simulink model "trt_model"  (R2025a)
settings: Solver=ode4  StartTime=0.0  StopTime=100  FixedStep=P.dt_sim  RelTol=1e-3
values from neighbouring files (symbols this model uses):
  C = aggressive_bypass_tuning(P, C, 0.3); end    [make_scenario.m]
  P = params()    [run_scenarios.m]
undefined symbols (not defined in the file or in its folder): X0
settings Model: Creator=andreazanelli  LastModifiedBy=andreazanelli
settings DataIOCC: SaveOutput=off  SignalLogging=off  SaveTime=off
settings DebuggingCC: AlgebraicLoopMsg=error

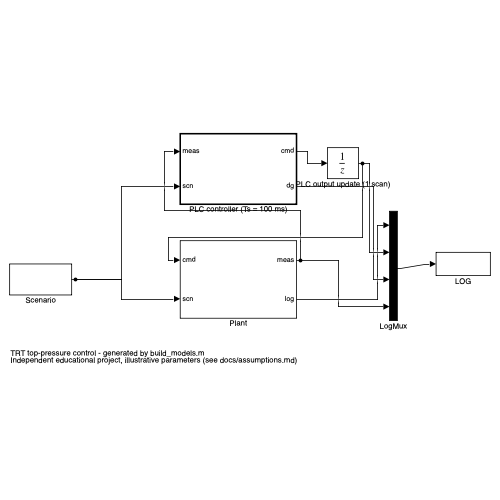
[thumbnail: Simulink's stored preview of the top-level diagram]
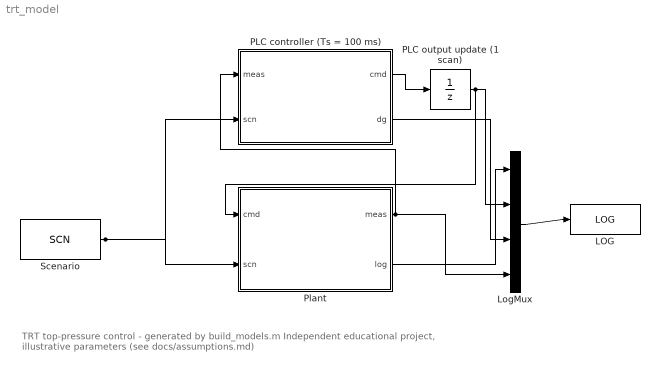
== system trt_model ==
  note: TRT top-pressure control - generated by build_models.m
      | Independent educational project, illustrative parameters (see docs/assumptions.md)
  LOG : ToWorkspace  VariableName=LOG  SaveFormat=Structure With Time  SampleTime=0.05
  LogMux : Mux
  PLC controller (Ts = 100 ms) : Subsystem  TreatAsAtomicUnit=on  SystemSampleTime=C.Ts
  PLC output update (1 scan) : UnitDelay  InitialCondition=C.init.cmd  SampleTime=C.Ts  HasFrameUpgradeWarning=on
  Plant : Subsystem
  Scenario : FromWorkspace  VariableName=SCN  SampleTime=C.Ts  Interpolate=off  OutputAfterFinalValue=Holding final value
  wires:
  Scenario/1 -> Plant/2(scn), PLC controller (Ts = 100 ms)/2(scn)
  PLC controller (Ts = 100 ms)/1(cmd) -> PLC output update (1 scan)/1
  PLC output update (1 scan)/1 -> Plant/1(cmd), LogMux/2
  Plant/1(meas) -> PLC controller (Ts = 100 ms)/1(meas), LogMux/4
  Plant/2(log) -> LogMux/1
  PLC controller (Ts = 100 ms)/2(dg) -> LogMux/3
  LogMux/1 -> LOG/1

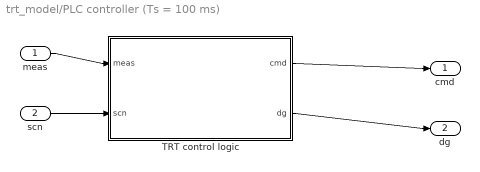
== system trt_model/PLC controller (Ts = 100 ms) ==
  meas : Inport
  scn : Inport  Port=2
  TRT control logic : MATLAB Function  TreatAsAtomicUnit=on
  cmd : Outport
  dg : Outport  Port=2
  wires:
  meas/1 -> TRT control logic/1(meas)
  scn/1 -> TRT control logic/2(scn)
  TRT control logic/1(cmd) -> cmd/1
  TRT control logic/2(dg) -> dg/1

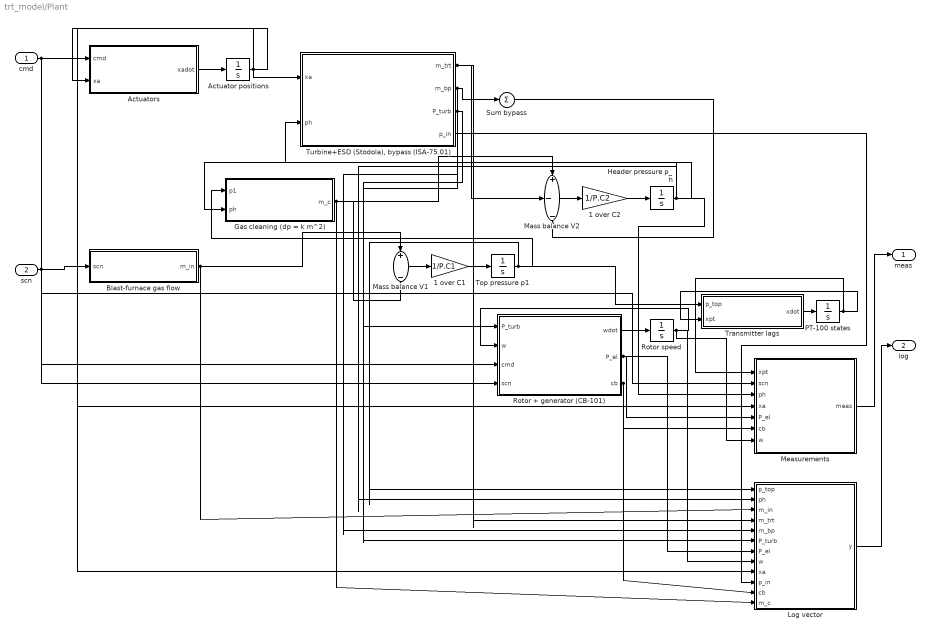
== system trt_model/Plant ==
  cmd : Inport
  scn : Inport  Port=2
  1 over C1 : Gain  Gain=1/P.C1
  1 over C2 : Gain  Gain=1/P.C2
  Actuator positions : Integrator  InitialCondition=X0.xa  LimitOutput=on  UpperSaturationLimit=1  LowerSaturationLimit=0
  Actuators : MATLAB Function  TreatAsAtomicUnit=on
  Blast-furnace gas flow : MATLAB Function  TreatAsAtomicUnit=on
  Gas cleaning (dp = k m^2) : MATLAB Function  TreatAsAtomicUnit=on
  Header pressure p_h : Integrator  InitialCondition=X0.ph
  Log vector : MATLAB Function  TreatAsAtomicUnit=on
  Mass balance V1 : Sum  Inputs=+-
  Mass balance V2 : Sum  Inputs=+--
  Measurements : MATLAB Function  TreatAsAtomicUnit=on
  PT-100 states : Integrator  InitialCondition=X0.xpt
  Rotor + generator (CB-101) : MATLAB Function  TreatAsAtomicUnit=on
  Rotor speed : Integrator  InitialCondition=X0.w
  Sum bypass : Sum  Inputs=+
  Top pressure p1 : Integrator  InitialCondition=X0.p1
  Transmitter lags : MATLAB Function  TreatAsAtomicUnit=on
  "Turbine+ESD (Stodola), bypass (ISA-75.01)" : MATLAB Function  TreatAsAtomicUnit=on
  meas : Outport
  log : Outport  Port=2
  wires:
  cmd/1 -> Actuators/1(cmd), Rotor + generator (CB-101)/3(cmd)
  Actuator positions/1 -> Actuators/2(xa), "Turbine+ESD (Stodola), bypass (ISA-75.01)"/1(xa), Measurements/4(xa), Log vector/9(xa)
  Actuators/1(xadot) -> Actuator positions/1
  Header pressure p_h/1 -> "Turbine+ESD (Stodola), bypass (ISA-75.01)"/2(ph), Gas cleaning (dp = k m^2)/2(ph), Measurements/3(ph), Log vector/2(ph)
  scn/1 -> Blast-furnace gas flow/1(scn), Rotor + generator (CB-101)/4(scn), Measurements/2(scn)
  Top pressure p1/1 -> Gas cleaning (dp = k m^2)/1(p1), Transmitter lags/1(p_top), Log vector/1(p_top)
  Blast-furnace gas flow/1(m_in) -> Mass balance V1/1, Log vector/3(m_in)
  Gas cleaning (dp = k m^2)/1(m_c) -> Mass balance V1/2, Mass balance V2/1, Log vector/12(m_c)
  Mass balance V1/1 -> 1 over C1/1
  1 over C1/1 -> Top pressure p1/1
  "Turbine+ESD (Stodola), bypass (ISA-75.01)"/1(m_trt) -> Mass balance V2/2, Log vector/4(m_trt)
  "Turbine+ESD (Stodola), bypass (ISA-75.01)"/2(m_bp) -> Sum bypass/1, Log vector/5(m_bp)
  Sum bypass/1 -> Mass balance V2/3
  Mass balance V2/1 -> 1 over C2/1
  1 over C2/1 -> Header pressure p_h/1
  "Turbine+ESD (Stodola), bypass (ISA-75.01)"/3(P_turb) -> Rotor + generator (CB-101)/1(P_turb), Log vector/6(P_turb)
  Rotor speed/1 -> Rotor + generator (CB-101)/2(w), Measurements/7(w), Log vector/8(w)
  Rotor + generator (CB-101)/1(wdot) -> Rotor speed/1
  PT-100 states/1 -> Transmitter lags/2(xpt), Measurements/1(xpt)
  Transmitter lags/1(xdot) -> PT-100 states/1
  Rotor + generator (CB-101)/2(P_el) -> Measurements/5(P_el), Log vector/7(P_el)
  Rotor + generator (CB-101)/3(cb) -> Measurements/6(cb), Log vector/11(cb)
  Measurements/1(meas) -> meas/1
  "Turbine+ESD (Stodola), bypass (ISA-75.01)"/4(p_in) -> Log vector/10(p_in)
  Log vector/1(y) -> log/1

== matlab function trt_model/PLC controller (Ts = 100 ms)/TRT control logic ==
  data: meas input; cmd output; scn input; dg output; C parameter
function [cmd, dg] = f(meas, scn, C)
[cmd, dg] = trt_controller_step(meas, scn, C);

== matlab function trt_model/Plant/Turbine+ESD (Stodola), bypass (ISA-75.01) ==
  data: xa input; m_trt output; ph input; m_bp output; P_turb output; p_in output; P parameter
function [m_trt, m_bp, P_turb, p_in] = f(xa, ph, P)
[m_trt, m_bp, P_turb, p_in] = plant_flows(xa, ph, P);

== matlab function trt_model/Plant/Actuators ==
  data: cmd input; xadot output; xa input; P parameter
function xadot = f(cmd, xa, P)
xadot = plant_actuators(cmd, xa, P);

== matlab function trt_model/Plant/Blast-furnace gas flow ==
  data: scn input; m_in output
function m_in = f(scn)
m_in = scn(1);

== matlab function trt_model/Plant/Gas cleaning (dp = k m^2) ==
  data: p1 input; m_c output; ph input; P parameter
function m_c = f(p1, ph, P)
m_c = plant_cleaning(p1, ph, P);

== matlab function trt_model/Plant/Rotor + generator (CB-101) ==
  data: P_turb input; wdot output; w input; cmd input; scn input; P_el output; cb output; P parameter
function [wdot, P_el, cb] = f(P_turb, w, cmd, scn, P)
[wdot, P_el, cb] = plant_rotor(P_turb, w, cmd, scn, P);

== matlab function trt_model/Plant/Transmitter lags ==
  data: p_top input; xdot output; xpt input; P parameter
function xdot = f(p_top, xpt, P)
xdot = (p_top - xpt) / P.pt.tau;

== matlab function trt_model/Plant/Measurements ==
  data: xpt input; meas output; scn input; ph input; xa input; P_el input; cb input; w input; P parameter
function meas = f(xpt, scn, ph, xa, P_el, cb, w, P)
meas = plant_meas(xpt, scn, ph, xa, P_el, cb, w, P);

== matlab function trt_model/Plant/Log vector ==
  data: p_top input; y output; ph input; m_in input; m_trt input; m_bp input; P_turb input; P_el input; w input; xa input; p_in input; cb input; m_c input
function y = f(p_top, ph, m_in, m_trt, m_bp, P_turb, P_el, w, xa, p_in, cb, m_c)
y = [p_top; ph; m_in; m_trt; m_bp(1); m_bp(2); P_turb; P_el; w; xa(1); xa(2); xa(3); xa(4); p_in; cb; m_c];
